simulink model "singele_phase_to_3phase_svpwm_PMSM_VF"  (R2025a)
settings: Solver=ode23t  StartTime=0.0  StopTime=5  FixedStep=0.00001  MaxStep=10e-6  RelTol=1e-3  EnableMultiTasking=on
undefined symbols (not defined in the file): F_cmd
libraries: spsSeriesRLCBranchLib x4, simulink x2, spsACVoltageSourceLib x1, spsGroundLib x1, spsPermanentMagnetSynchronousMachineLib x1, spsThreeLevelBridgeLib x1, spsThreePhaseVIMeasurementLib x1, spsUniversalBridgeLib x1, spsVoltageMeasurementLib x1, spspowerguiLib x1
settings Model: Creator=jagan  LastModifiedBy=SimuVerity Contributors
settings SolverCC: ZeroCrossControl=DisableAll  ZeroCrossAlgorithm=Non-adaptive  AlgebraicLoopSolver=TrustRegion
settings DataIOCC: LimitDataPoints=on  SaveFormat=Array  SignalLoggingSaveFormat=ModelDataLogs  ReturnWorkspaceOutputs=off
settings OptimizationCC: ExpressionDepthLimit=2147483647.0  InitFltsAndDblsToZero=on  LifeSpan=inf
settings DebuggingCC: SaveWithParameterizedLinksMsg=none  UnderspecifiedInitializationDetection=Classic  MergeDetectMultiDrivingBlocksExec=none  SignalResolutionControl=TryResolveAllWithWarning  SolverPrmCheckMsg=warning  MultiTaskDSMMsg=warning  MultiTaskCondExecSysMsg=none  FcnCallInpInsideContextMsg=warning  UnconnectedInputMsg=warning  UnconnectedOutputMsg=warning  UnconnectedLineMsg=warning  StateNameClashWarn=warning  SFUnexpectedBacktrackingDiag=warning  SFNoUnconditionalDefaultTransitionDiag=warning  SFExecutionAtInitializationDiag=none  ArithmeticOperatorsInVariantConditions=warning
settings HardwareCC: ProdBitPerPointer=32.0  ProdBitPerSizeT=32.0  ProdBitPerPtrDiffT=32.0  ProdLargestAtomicFloat=None  ProdIntDivRoundTo=Undefined  ProdEndianess=Unspecified  ProdWordSize=32.0  ProdHWDeviceType=32-bit Generic
settings ModelReferenceCC: PropagateSignalLabelsOutOfModel=off
settings SFSimCC: SimParseCustomCode=off
settings RTWCC: GPUComputeCapability=3.5
settings CodeAppCC: StateflowObjectComments=on
settings GRTTargetCC: TargetFcnLib=ansi_tfl_tmw.mat  TargetLangStandard=C89/C90 (ANSI)  CombineOutputUpdateFcns=off  GRTInterface=on
settings ConfigComp: CovMetricSettings=dw  CovSaveCumulativeToWorkspaceVar=on  CovSaveSingleToWorkspaceVar=on

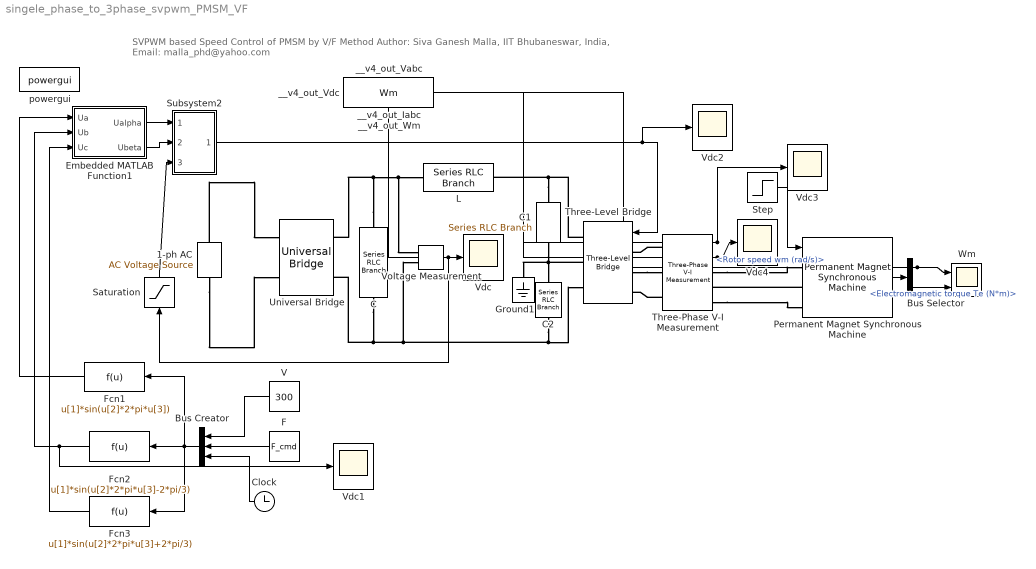
== system singele_phase_to_3phase_svpwm_PMSM_VF ==
  note: SVPWM based  Speed Control  of PMSM by V/F Method
      | Author: Siva Ganesh Malla, IIT Bhubaneswar, India, Email: malla_phd@yahoo.com
  1-ph AC : spsACVoltageSourceLib/AC Voltage Source  Amplitude=650  Phase=0  Frequency=50  SampleTime=0  Measurements=None  BusType=swing  Pref=10e3  Qref=0  Qmin=-inf  Qmax=+inf
  Bus Creator : BusCreator  Inputs=3
  Bus Selector : BusSelector  OutputSignals=Rotor speed wm (rad/s),Electromagnetic torque Te (N*m)
  C : spsSeriesRLCBranchLib/Series RLC Branch  LConnTagsString=__new0  RConnTagsString=__new0  BranchType=C  Resistance=1  Inductance=1e-3  SetiL0=off  InitialCurrent=0  Capacitance=10e-6  Setx0=off  InitialVoltage=0  Measurements=None
  C1 : spsSeriesRLCBranchLib/Series RLC Branch  LConnTagsString=__new0  RConnTagsString=__new0  BranchType=C  Resistance=1  Inductance=1e-3  SetiL0=off  InitialCurrent=0  Capacitance=2300e-6  Setx0=off  InitialVoltage=0  Measurements=None
  C2 : spsSeriesRLCBranchLib/Series RLC Branch  LConnTagsString=__new0  RConnTagsString=__new0  BranchType=C  Resistance=1  Inductance=1e-3  SetiL0=off  InitialCurrent=0  Capacitance=2300e-6  Setx0=off  InitialVoltage=0  Measurements=None
  Clock : Clock
  Embedded MATLAB Function1 : MATLAB Function  TreatAsAtomicUnit=on
  F : Constant  Value=F_cmd
  Fcn1 : Fcn  Expr=u[1]*sin(u[2]*2*pi*u[3])
  Fcn2 : Fcn  Expr=u[1]*sin(u[2]*2*pi*u[3]-2*pi/3)
  Fcn3 : Fcn  Expr=u[1]*sin(u[2]*2*pi*u[3]+2*pi/3)
  Ground1 : spsGroundLib/Ground  LConnTagsString=a
  L : spsSeriesRLCBranchLib/Series RLC Branch  LConnTagsString=__new0  RConnTagsString=__new0  BranchType=L  Resistance=1  Inductance=0.1e-3  SetiL0=off  InitialCurrent=0  Capacitance=1e-6  Setx0=off  InitialVoltage=0  Measurements=None
  Permanent Magnet Synchronous Machine : spsPermanentMagnetSynchronousMachineLib/Permanent Magnet Synchronous Machine  NbPhases=3  FluxDistribution=Sinusoidal  RotorType=Salient-pole  MechanicalLoad=Torque Tm  PresetModel=No  ShowDetailedParameters=on  MeasurementBus=off  Resistance=18.7  Inductance=8.5e-3  dqInductances=[0.02682 0.02682]  La=0.000395  MachineConstant=Flux linkage established by magnets (V.s)  Flux=0.1717  VoltageCst=62.2859  TorqueCst=0.5151  Flat=120  Mechanical=[2.26e-005 1.349e-005 2]  PolePairs=2  InitialConditions=[0,0, 0,0]  InitialConditions5ph=[0 0 0 0 0 0]  RefAngle=90 degrees behind phase A axis (modified Park)  IterativeDiscreteModel=Trapezoidal non iterative  TsBlock=-1  TsPowergui=0
  Saturation : Saturate  UpperLimit=750  LowerLimit=10
  Step : Step  After=3  SampleTime=0
  Subsystem2 : Subsystem
  Three-Level Bridge : spsThreeLevelBridgeLib/Three-Level Bridge  Arms=3  SnubberResistance=50  SbubberCapacitance=1e-6  Device=IGBT / Diodes  Ron=0.2e-3  ForwardVoltages="[  2 1 ]"  Measurements=All voltages and currents
      settings: AttributesFormatString=\n  LibrarySourceBlock=sps_lib/Power Electronics/Three-Level Bridge
  Three-Phase V-I Measurement : spsThreePhaseVIMeasurementLib/Three-Phase V-I Measurement  VoltageMeasurement=phase-to-phase  SetLabelV=off  LabelV=Vabc  Vpu=off  VpuLL=off  CurrentMeasurement=yes  SetLabelI=off  LabelI=Iabc  Ipu=off  Pbase=100e6  Vbase=500e3  OutputType=Complex  PhasorSimulation=off  PSBequivalent=0
  Universal Bridge : spsUniversalBridgeLib/Universal Bridge  Arms=2  SnubberResistance=1e5  SnubberCapacitance=inf  Device=Diodes  Ron=1e-3  Lon=0  ForwardVoltages="[  0  0  ]"  ForwardVoltage=0  GTOparameters=[ 10e-6 , 20e-6 ]  IGBTparameters=[ 1e-6 , 2e-6 ]  Measurements=None  Measurements_2=None  converterType=Rectifier
  V : Constant  Value=300
  Vdc{,1..4} (5 alike) : Scope
      Vdc settings: SampleTime=100e-6  TimeSpan=1  ActiveDisplayYMinimum=225  ActiveDisplayYMaximum=750  DataLoggingVariableName=Ia_
      Vdc1 settings: SampleTime=100e-6  TimeSpan=1  ActiveDisplayYMinimum=-400  ActiveDisplayYMaximum=400  DataLoggingVariableName=Ia_1
      Vdc2 settings: SampleTime=100e-6  TimeSpan=1  ActiveDisplayYMinimum=0  ActiveDisplayYMaximum=1  DataLoggingVariableName=Ia_2
      Vdc3 settings: SampleTime=100e-6  TimeSpan=0.04  ActiveDisplayYMinimum=-700  ActiveDisplayYMaximum=700  DataLoggingVariableName=Ia_3
      Vdc4 settings: SampleTime=100e-6  TimeSpan=1  ActiveDisplayYMinimum=-90  ActiveDisplayYMaximum=90  DataLoggingVariableName=Ia_4
  Voltage Measurement : spsVoltageMeasurementLib/Voltage Measurement  PhasorSimulation=off  OutputType=Complex  PSBequivalent=0
  Wm : Scope  NumInputPorts=2
      settings: ActiveDisplayYMinimum=135  ActiveDisplayYMaximum=182.5  DataLoggingVariableName=ScopeData9
  __v4_out_Iabc : ToWorkspace  VariableName=Iabc  SaveFormat=Timeseries  SampleTime=-1
  __v4_out_Vabc : ToWorkspace  VariableName=Vabc  SaveFormat=Timeseries  SampleTime=-1
  __v4_out_Vdc : ToWorkspace  VariableName=Vdc  SaveFormat=Timeseries  SampleTime=-1
  __v4_out_Wm : ToWorkspace  VariableName=Wm  SaveFormat=Timeseries  SampleTime=-1
  powergui : spspowerguiLib/powergui  SimulationMode=Discrete  SampleTime=50e-6  frequency=60  Iterations=50  frequencyindice=50  Pbase=100e6  ErrMax=1e-4  UnitsV=kV  UnitsW=MW  buscounter=0  FunctionMessages=off  echomessages=off  EnableUseOfTLC=off  CurrentSourceSwitches=off  DisableSnubberDevices=off  DisableRonSwitches=off  DisableVfSwitches=off  DisplayEquations=off  AutomaticDiscreteSolvers=off  SolverType=Tustin/Backward Euler (TBE)  Interpol=off  ExternalGateDelay=off  methode=off  Ts=0  x0status=blocks  SPID=off  SwTol=0  HookPort=off  NonlinearTolerance=1e-4  nMaxIteration=100  ContinueOnMaxIteration=off  RestoreLinks=warning  ResistiveCurrentMeasurement=off  Frange=[0:2:500]  Ylog=off  Xlog=on  ShowGrid=off  save=off  variable=ZData  structure=0  ZoomFFT=on  StartTime=0.0  cycles=1  DisplayStyle=1  fundamental=60  FreqAxis=off  MaxFrequency=1000  frequencyindicesteady=1  RmsSteady=1  display=off
  wires:
  Step/1 -> Permanent Magnet Synchronous Machine/1
  Embedded MATLAB Function1/1(Ualpha) -> Subsystem2/1(Ualfa)
  Embedded MATLAB Function1/2(Ubeta) -> Subsystem2/2(Ubeta)
  Permanent Magnet Synchronous Machine/1 -> Bus Selector/1
  Bus Selector/1 -> Wm/1, __v4_out_Wm/1  "<Rotor speed wm (rad/s)>"
  Bus Selector/2 -> Wm/2  "<Electromagnetic torque Te (N*m)>"
  Subsystem2/1(pulse) -> Three-Level Bridge/1, Vdc2/1
  Three-Phase V-I Measurement/1 -> Vdc3/1, __v4_out_Vabc/1
  Three-Phase V-I Measurement/2 -> Vdc4/1, __v4_out_Iabc/1
  Bus Creator/1 -> Fcn2/1, Fcn1/1, Fcn3/1
  Clock/1 -> Bus Creator/3
  Fcn1/1 -> Embedded MATLAB Function1/1(Ua)
  Fcn2/1 -> Embedded MATLAB Function1/2(Ub), Vdc1/1
  Fcn3/1 -> Embedded MATLAB Function1/3(Uc)
  Voltage Measurement/1 -> Vdc/1, Saturation/1, __v4_out_Vdc/1
  Saturation/1 -> Subsystem2/3(Vdc)
  V/1 -> Bus Creator/1
  F/1 -> Bus Creator/2
  connections:
  Three-Phase V-I Measurement/LConn1 -- Three-Level Bridge/LConn1
  Three-Level Bridge/LConn2 -- Three-Phase V-I Measurement/LConn2
  Three-Phase V-I Measurement/LConn3 -- Three-Level Bridge/LConn3
  Three-Phase V-I Measurement/RConn1 -- Permanent Magnet Synchronous Machine/LConn1
  Permanent Magnet Synchronous Machine/LConn2 -- Three-Phase V-I Measurement/RConn2
  Three-Phase V-I Measurement/RConn3 -- Permanent Magnet Synchronous Machine/LConn3
  C/LConn1 -- L/LConn1 -- Voltage Measurement/LConn1 -- Universal Bridge/RConn1
  Three-Level Bridge/RConn3 -- C2/RConn1 -- Voltage Measurement/LConn2 -- Universal Bridge/RConn2 -- C/RConn1
  C1/LConn1 -- Three-Level Bridge/RConn1 -- L/RConn1
  Ground1/LConn1 -- C1/RConn1 -- C2/LConn1 -- Three-Level Bridge/RConn2
  1-ph AC/RConn1 -- Universal Bridge/LConn1
  1-ph AC/LConn1 -- Universal Bridge/LConn2

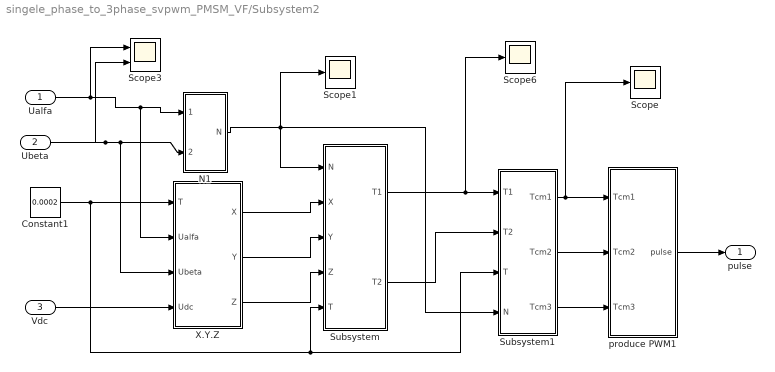
== system singele_phase_to_3phase_svpwm_PMSM_VF/Subsystem2 ==
  Ualfa : Inport
  Ubeta : Inport  Port=2
  Vdc : Inport  Port=3
  Constant1 : Constant  Value=0.0002
  N1 : Subsystem
  Scope : Scope
      settings: TimeSpan=0.4  ActiveDisplayYMinimum=2E-5  ActiveDisplayYMaximum=8E-5
  Scope1 : Scope
      settings: ActiveDisplayYMinimum=2  ActiveDisplayYMaximum=6
  Scope3 : Scope  NumInputPorts=2
      settings: TimeSpan=0.1  ActiveDisplayYMinimum=7.5  ActiveDisplayYMaximum=37.5  DataLoggingVariableName=ScopeData2
  Scope6 : Scope
      settings: ActiveDisplayYMinimum=2  ActiveDisplayYMaximum=6  DataLoggingVariableName=ScopeData3
  Subsystem : Subsystem
  Subsystem1 : Subsystem
  X.Y.Z : Subsystem
  produce PWM1 : Subsystem
  pulse : Outport
  wires:
  Constant1/1 -> X.Y.Z/1(T), Subsystem1/3(T), Subsystem/5(T)
  Vdc/1 -> X.Y.Z/4(Udc)
  N1/1(N) -> Subsystem1/4(N), Scope1/1, Subsystem/1(N)
  X.Y.Z/1(X) -> Subsystem/2(X)
  X.Y.Z/2(Y) -> Subsystem/3(Y)
  X.Y.Z/3(Z) -> Subsystem/4(Z)
  Subsystem1/1(Tcm1) -> Scope/1, produce PWM1/1(Tcm1)
  Subsystem1/2(Tcm2) -> produce PWM1/2(Tcm2)
  Subsystem1/3(Tcm3) -> produce PWM1/3(Tcm3)
  Ualfa/1 -> Scope3/1, X.Y.Z/2(Ualfa), N1/1(Ualfa)
  Subsystem/1(T1) -> Subsystem1/1(T1), Scope6/1
  Subsystem/2(T2) -> Subsystem1/2(T2)
  Ubeta/1 -> N1/2(Ubeta), X.Y.Z/3(Ubeta), Scope3/2
  produce PWM1/1(pulse) -> pulse/1

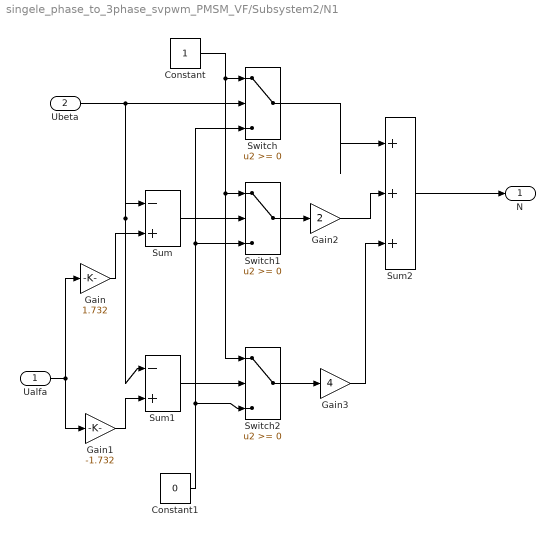
== system singele_phase_to_3phase_svpwm_PMSM_VF/Subsystem2/N1 ==
  Ualfa : Inport
  Ubeta : Inport  Port=2
  Constant : Constant
  Constant1 : Constant  Value=0
  Gain : Gain  Gain=1.732
  Gain1 : Gain  Gain=-1.732
  Gain2 : Gain  Gain=2
  Gain3 : Gain  Gain=4
  Sum : Sum  Inputs=|-+
  Sum1 : Sum  Inputs=|-+
  Sum2 : Sum  Inputs=|+++
  Switch : Switch  SaturateOnIntegerOverflow=off  InputSameDT=off
  Switch1 : Switch  SaturateOnIntegerOverflow=off  InputSameDT=off
  Switch2 : Switch  SaturateOnIntegerOverflow=off  InputSameDT=off
  N : Outport
  wires:
  Ubeta/1 -> Switch/2, Sum/1, Sum1/1
  Constant/1 -> Switch/1, Switch2/1, Switch1/1
  Ualfa/1 -> Gain1/1, Gain/1
  Gain/1 -> Sum/2
  Sum/1 -> Switch1/2
  Sum1/1 -> Switch2/2
  Gain1/1 -> Sum1/2
  Constant1/1 -> Switch/3, Switch1/3, Switch2/3
  Switch1/1 -> Gain2/1
  Switch2/1 -> Gain3/1
  Gain2/1 -> Sum2/2
  Switch/1 -> Sum2/1
  Gain3/1 -> Sum2/3
  Sum2/1 -> N/1

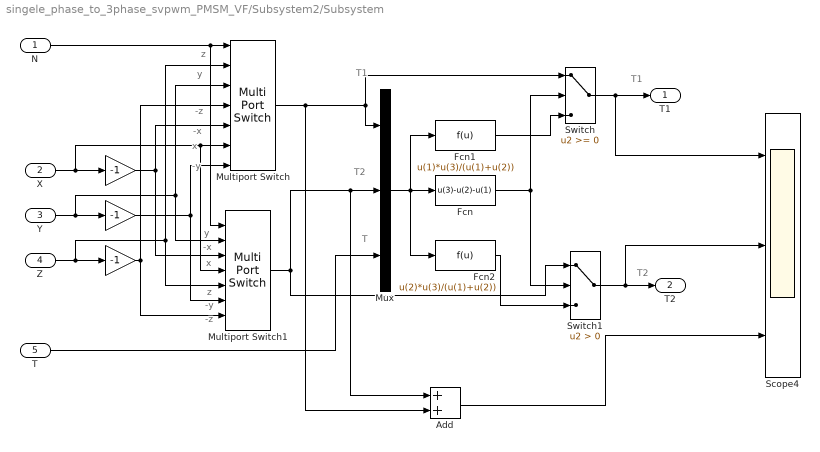
== system singele_phase_to_3phase_svpwm_PMSM_VF/Subsystem2/Subsystem ==
  note: z
  note: y
  note: -z
  note: -x
  note: x
  note: -y
  note: y
  note: -x
  note: x
  note: z
  note: -y
  note: -z
  note: T1
  note: T2
  note: T
  note: T1
  note: T2
  N : Inport
  X : Inport  Port=2
  Y : Inport  Port=3
  Z : Inport  Port=4
  T : Inport  Port=5
  " " : Gain  Gain=-1
  "  " : Gain  Gain=-1
  "    " : Gain  Gain=-1
  Add : Sum
  Fcn : Fcn  Expr=u(3)-u(2)-u(1)
  Fcn1 : Fcn  Expr=u(1)*u(3)/(u(1)+u(2))
  Fcn2 : Fcn  Expr=u(2)*u(3)/(u(1)+u(2))
  Multiport Switch : MultiPortSwitch  Inputs=6  SaturateOnIntegerOverflow=off  InputSameDT=off
  Multiport Switch1 : MultiPortSwitch  Inputs=6  SaturateOnIntegerOverflow=off  InputSameDT=off
  Mux : Mux  Inputs=3
  Scope4 : Scope  NumInputPorts=3
      settings: TimeSpan=0.35  ActiveDisplayYMinimum=-1E-5  ActiveDisplayYMaximum=0.00018  DataLoggingVariableName=ScopeData4
  Switch : Switch  SaturateOnIntegerOverflow=off  InputSameDT=off
  Switch1 : Switch  Criteria=u2 > Threshold  SaturateOnIntegerOverflow=off  InputSameDT=off
  T1 : Outport
  T2 : Outport  Port=2
  wires:
  N/1 -> Multiport Switch1/1, Multiport Switch/1
  X/1 -> Multiport Switch1/4, Multiport Switch/6, " "/1
  Y/1 -> Multiport Switch1/2, Multiport Switch/3, "  "/1
  Z/1 -> Multiport Switch1/5, Multiport Switch/2, "    "/1
  "    "/1 -> Multiport Switch1/7, Multiport Switch/4
  "  "/1 -> Multiport Switch/7, Multiport Switch1/6
  " "/1 -> Multiport Switch/5, Multiport Switch1/3
  Multiport Switch/1 -> Mux/1, Switch/1, Add/2
  Multiport Switch1/1 -> Switch1/1, Mux/2, Add/1
  T/1 -> Mux/3
  Mux/1 -> Fcn/1, Fcn1/1, Fcn2/1
  Fcn/1 -> Switch/2, Switch1/2
  Fcn1/1 -> Switch/3
  Fcn2/1 -> Switch1/3
  Switch/1 -> T1/1, Scope4/1
  Switch1/1 -> T2/1, Scope4/2
  Add/1 -> Scope4/3

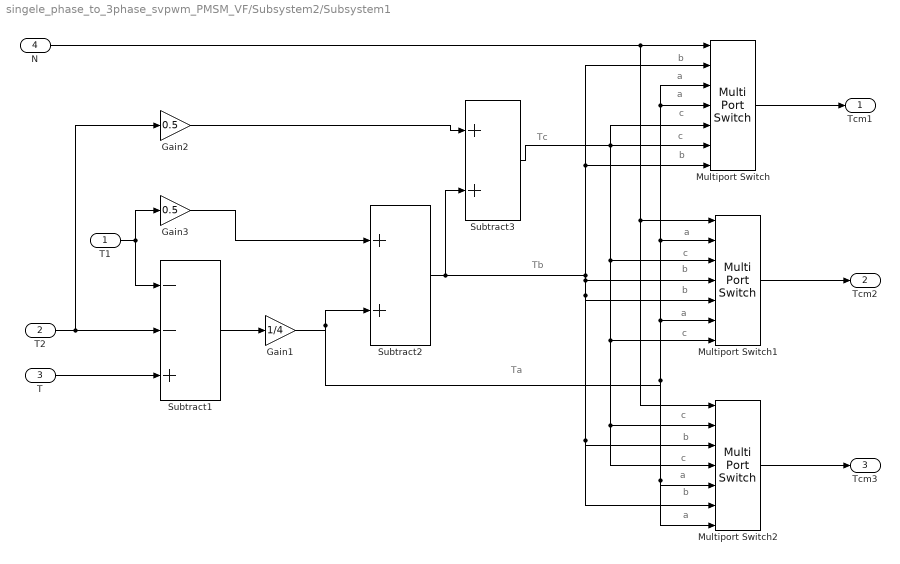
== system singele_phase_to_3phase_svpwm_PMSM_VF/Subsystem2/Subsystem1 ==
  note: Ta
  note: Tb
  note: Tc
  note: b
  note: a
  note: a
  note: c
  note: c
  note: b
  note: a
  note: c
  note: b
  note: b
  note: a
  note: c
  note: c
  note: b
  note: c
  note: a
  note: b
  note: a
  T1 : Inport
  T2 : Inport  Port=2
  T : Inport  Port=3
  N : Inport  Port=4
  Gain1 : Gain  Gain=1/4
  Gain2 : Gain  Gain=0.5
  Gain3 : Gain  Gain=0.5
  Multiport Switch : MultiPortSwitch  Inputs=6  SaturateOnIntegerOverflow=off  InputSameDT=off
  Multiport Switch1 : MultiPortSwitch  Inputs=6  SaturateOnIntegerOverflow=off  InputSameDT=off
  Multiport Switch2 : MultiPortSwitch  Inputs=6  SaturateOnIntegerOverflow=off  InputSameDT=off
  Subtract1 : Sum  Inputs=--+
  Subtract2 : Sum
  Subtract3 : Sum
  Tcm1 : Outport
  Tcm2 : Outport  Port=2
  Tcm3 : Outport  Port=3
  wires:
  T2/1 -> Gain2/1, Subtract1/2
  T/1 -> Subtract1/3
  T1/1 -> Gain3/1, Subtract1/1
  Gain3/1 -> Subtract2/1
  Subtract1/1 -> Gain1/1
  Gain1/1 -> Subtract2/2, Multiport Switch/3, Multiport Switch/4, Multiport Switch1/2, Multiport Switch1/6, Multiport Switch2/5, Multiport Switch2/7
  Subtract2/1 -> Subtract3/2, Multiport Switch/2, Multiport Switch/7, Multiport Switch1/4, Multiport Switch1/5, Multiport Switch2/3, Multiport Switch2/6
  Gain2/1 -> Subtract3/1
  N/1 -> Multiport Switch/1, Multiport Switch2/1, Multiport Switch1/1
  Multiport Switch/1 -> Tcm1/1
  Multiport Switch1/1 -> Tcm2/1
  Multiport Switch2/1 -> Tcm3/1
  Subtract3/1 -> Multiport Switch/5, Multiport Switch/6, Multiport Switch1/3, Multiport Switch1/7, Multiport Switch2/2, Multiport Switch2/4

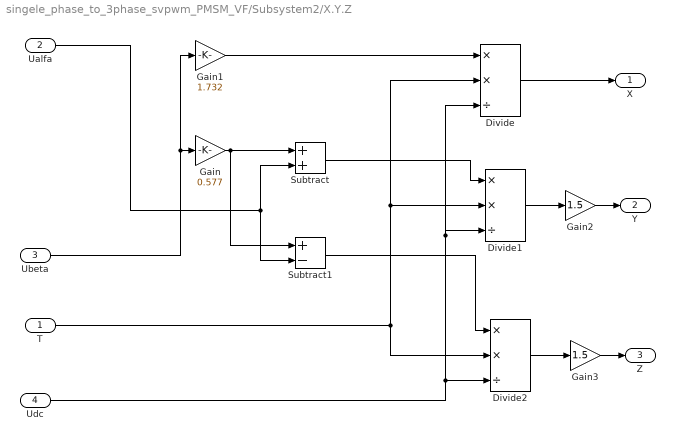
== system singele_phase_to_3phase_svpwm_PMSM_VF/Subsystem2/X.Y.Z ==
  T : Inport
  Ualfa : Inport  Port=2
  Ubeta : Inport  Port=3
  Udc : Inport  Port=4
  Divide : Product  Inputs=**/
  Divide1 : Product  Inputs=**/
  Divide2 : Product  Inputs=**/
  Gain : Gain  Gain=0.577
  Gain1 : Gain  Gain=1.732
  Gain2 : Gain  Gain=1.5
  Gain3 : Gain  Gain=1.5
  Subtract : Sum
  Subtract1 : Sum  Inputs=+-
  X : Outport
  Y : Outport  Port=2
  Z : Outport  Port=3
  wires:
  Gain/1 -> Subtract/1, Subtract1/1
  Gain1/1 -> Divide/1
  T/1 -> Divide2/2, Divide1/2, Divide/2
  Udc/1 -> Divide2/3, Divide1/3, Divide/3
  Ualfa/1 -> Subtract1/2, Subtract/2
  Subtract/1 -> Divide1/1
  Subtract1/1 -> Divide2/1
  Divide/1 -> X/1
  Divide1/1 -> Gain2/1
  Divide2/1 -> Gain3/1
  Gain2/1 -> Y/1
  Gain3/1 -> Z/1
  Ubeta/1 -> Gain1/1, Gain/1

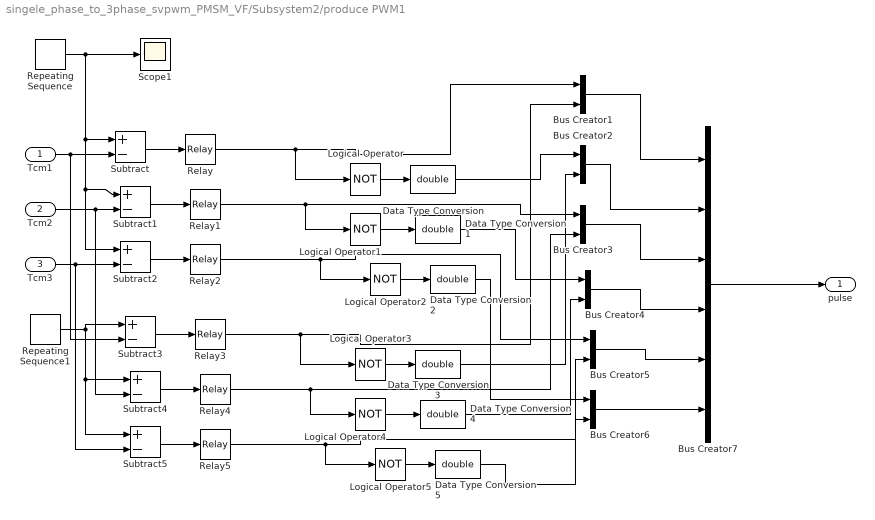
== system singele_phase_to_3phase_svpwm_PMSM_VF/Subsystem2/produce PWM1 ==
  Tcm1 : Inport
  Tcm2 : Inport  Port=2
  Tcm3 : Inport  Port=3
  Bus Creator{1..6} (6 alike) : BusCreator  Inputs=2
  Bus Creator7 : BusCreator  Inputs=6
  Data Type Conversion{,1..5} (6 alike) : DataTypeConversion  OutDataTypeStr=double  SaturateOnIntegerOverflow=off  RndMeth=Floor
  Logical Operator{,1..5} (6 alike) : Logic  Operator=NOT  AllPortsSameDT=off
  Relay{,1..5} (6 alike) : Relay
  Repeating Sequence : simulink/Sources/Repeating Sequence  rep_seq_t=[0 0.0001 0.0002]  rep_seq_y=[0 0.0001/2 0]
  Repeating Sequence1 : simulink/Sources/Repeating Sequence  rep_seq_t=[0 0.0001 0.0002]  rep_seq_y=[0.0001/2 0.0001 0.0001/2]
  Scope1 : Scope
      settings: TimeSpan=1  ActiveDisplayYMinimum=-0.0025  ActiveDisplayYMaximum=0.004  DataLoggingVariableName=ScopeData6
  Subtract{,1..5} (6 alike) : Sum  Inputs=+-
  pulse : Outport
  wires:
  Data Type Conversion2/1 -> Bus Creator6/1
  Data Type Conversion1/1 -> Bus Creator4/1
  Data Type Conversion/1 -> Bus Creator2/1
  Relay2/1 -> Logical Operator2/1, Bus Creator5/1
  Relay1/1 -> Logical Operator1/1, Bus Creator3/1
  Relay/1 -> Logical Operator/1, Bus Creator1/1
  Logical Operator/1 -> Data Type Conversion/1
  Logical Operator2/1 -> Data Type Conversion2/1
  Logical Operator1/1 -> Data Type Conversion1/1
  Tcm3/1 -> Subtract2/2, Subtract5/2
  Tcm2/1 -> Subtract1/2, Subtract4/2
  Tcm1/1 -> Subtract/2, Subtract3/2
  Repeating Sequence/1 -> Scope1/1, Subtract1/1, Subtract2/1, Subtract/1
  Subtract2/1 -> Relay2/1
  Subtract1/1 -> Relay1/1
  Subtract/1 -> Relay/1
  Subtract5/1 -> Relay5/1
  Subtract4/1 -> Relay4/1
  Subtract3/1 -> Relay3/1
  Repeating Sequence1/1 -> Subtract3/1, Subtract4/1, Subtract5/1
  Data Type Conversion5/1 -> Bus Creator6/2
  Data Type Conversion4/1 -> Bus Creator4/2
  Data Type Conversion3/1 -> Bus Creator2/2
  Relay5/1 -> Logical Operator5/1, Bus Creator5/2
  Relay4/1 -> Logical Operator4/1, Bus Creator3/2
  Relay3/1 -> Logical Operator3/1, Bus Creator1/2
  Logical Operator3/1 -> Data Type Conversion3/1
  Logical Operator5/1 -> Data Type Conversion5/1
  Logical Operator4/1 -> Data Type Conversion4/1
  Bus Creator1/1 -> Bus Creator7/1
  Bus Creator2/1 -> Bus Creator7/2
  Bus Creator3/1 -> Bus Creator7/3
  Bus Creator4/1 -> Bus Creator7/4
  Bus Creator5/1 -> Bus Creator7/5
  Bus Creator6/1 -> Bus Creator7/6
  Bus Creator7/1 -> pulse/1

== matlab function singele_phase_to_3phase_svpwm_PMSM_VF/Embedded MATLAB Function1 ==
  settings: fimath=|
      | fimath(...
      | 'RoundMode', 'floor',...
      | 'OverflowMode', 'wrap',...
      | 'ProductMode', 'KeepLSB', 'ProductWordLength', 32,...
      | 'SumMode', 'KeepLSB', 'SumWordLength', 32,...
      | 'CastBeforeSum', false)
  data: Ua input; Ualpha output; Ub input; Uc input; Ubeta output
function [Ualpha,Ubeta]= fcn(Ua,Ub,Uc)
% This block supports an embeddable subset of the MATLAB language.
% See the help menu for details. 

Ualpha=2/3*(Ua-0.5*Ub-0.5*Uc);
Ubeta=2/3*(sqrt(3)/2*Ub-sqrt(3)/2*Uc);
